simulink model "PV_CHAR"  (R2024a)
settings: Solver=VariableStepAuto  StartTime=0.0  StopTime=5  RelTol=1e-3
libraries: spsDiodeLib x12, spsPVArrayLib x12, spsControlledVoltageSourceLib x2, spsCurrentMeasurementLib x2, simulink x2, spsVoltageMeasurementLib x2, spspowerguiLib x1
settings Model: Creator=sarve  LastModifiedBy=Aswin

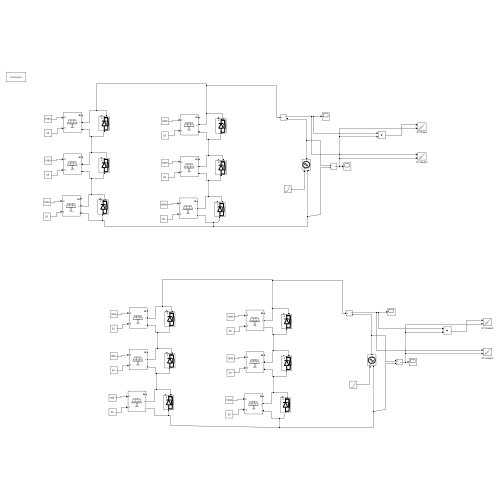
[thumbnail: Simulink's stored preview of the top-level diagram]
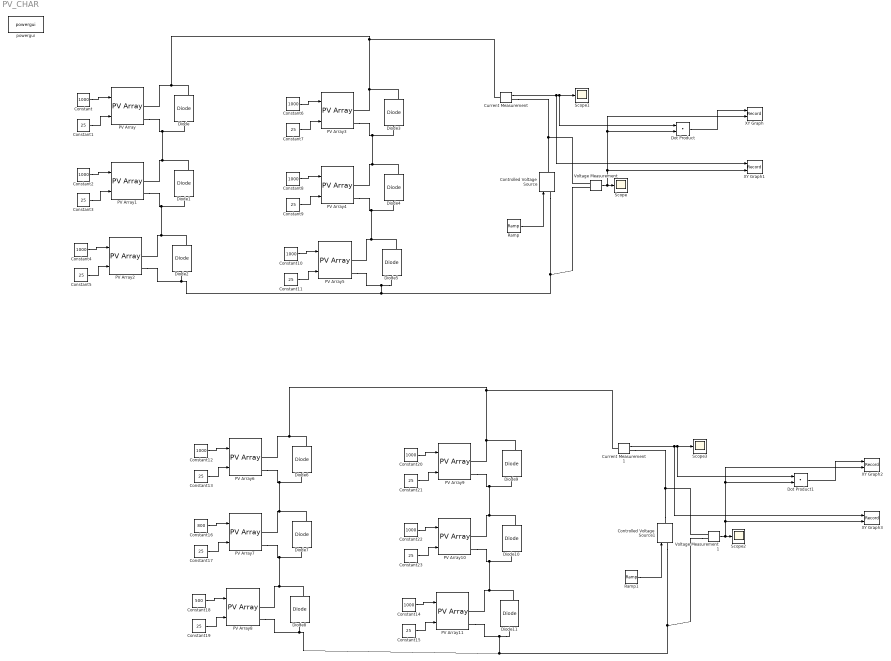
== system PV_CHAR ==
  Constant{,2,4,6,8,10,12,14,20,22} (10 alike) : Constant  Value=1000
  Constant{1,3,5,7,9,11,13,15,17,19,21,23} (12 alike) : Constant  Value=25
  Constant16 : Constant  Value=800
  Constant18 : Constant  Value=500
  Controlled Voltage Source : spsControlledVoltageSourceLib/Controlled Voltage Source  Initialize=on  Source_Type=AC  Amplitude=0  Phase=0  Frequency=0  Measurements=None
  Controlled Voltage Source1 : spsControlledVoltageSourceLib/Controlled Voltage Source  Initialize=on  Source_Type=AC  Amplitude=0  Phase=0  Frequency=0  Measurements=None
  Current Measurement : spsCurrentMeasurementLib/Current Measurement  PhasorSimulation=off  OutputType=Complex  PSBequivalent=0
  Current Measurement1 : spsCurrentMeasurementLib/Current Measurement  PhasorSimulation=off  OutputType=Complex  PSBequivalent=0
  Diode{,1..11} (12 alike) : spsDiodeLib/Diode  Ron=0.001  Lon=0  Vf=0.8  IC=0  UseSnubber=0  Rs=500  Cs=250e-9  Measurements=on
  Dot Product : DotProduct  OutDataTypeStr=Inherit: Inherit via internal rule
  Dot Product1 : DotProduct  OutDataTypeStr=Inherit: Inherit via internal rule
  PV Array{,1..11} (12 alike) : spsPVArrayLib/PV Array  Npar=40  Nser=10  PlotType=array @ 1000 W/m2 & specified temperatures  S_vec="[ 1000  500  100 ]"  Temp_C_vec="[ 45 25  ]"  ModuleName=User-defined  PlotWhenSelected=off  Pm=213.15  Ncell=60  Voc=36.3  Isc=7.84  Vm=29  Im=7.35  beta_Voc_pc=-0.36099  alpha_Isc_pc=0.102  beta_Voc=-0.13104  alpha_Isc=0.0079968  IL=7.8654  I0=2.9273e-10  nI=0.98119  Rsh=313.0553  Rs=0.39381  RobustModel=off  RobustCellTemperature=313.3991  BAL=on  Tc=1e-6  Tfilter=5e-5
  Ramp : simulink/Sources/Ramp  slope=36.3*3*2  start=0  InitialOutput=0
  Ramp1 : simulink/Sources/Ramp  slope=36.3*3*2  start=0  InitialOutput=0
  Scope{,1..3} (4 alike) : Scope
  Voltage Measurement : spsVoltageMeasurementLib/Voltage Measurement  PhasorSimulation=off  OutputType=Complex  PSBequivalent=0
  Voltage Measurement1 : spsVoltageMeasurementLib/Voltage Measurement  PhasorSimulation=off  OutputType=Complex  PSBequivalent=0
  XY Graph : Record  FileSettingsInternal="{\"entries\":[{\"content\":{\"excelSettings\":{\"content\":{},\"type\":\"Streamout.ExcelSettings\"}},\"type\":\"Streamout.FileSettingStorage\",\"uuid\":\"\"}],\"packageUris\":[\"http:\\/\\/schema.mathworks.com\\/mf0\\/streamout_blocks\\/R2020a\"],\"version\":\"1.0\"}"  Layout=[1 1]  SignalsInternal="{\"entries\":[{\"content\":{\"signals\":[{\"content\":{\"blockPath\":[],\"dimensions\":[1],\"domain\":\"\",\"lineColor\":\"#64d413\",\"lineWidth\":2,\"plots\":[ 1 ],\"port\":1,\"signalID\":1,\"signalName\":\"Dot Product\"},\"type\":\"RecordBlkView.Signal\",\"uuid\":\"\"},{\"content\":{\"blockPath\":[],\"dimensions\":[1],\"domain\":\"\",\"lineColor\":\"#ff13a6\",\"lineWidth\":2,\"plots\":[ 1 ],\"port\":2,\"signalID\":2,\"signalName\":\"Voltage Measurement\"},\"type\":\"RecordBlkView.Signal\",\"uuid\":\"\"}]},\"type\":\"RecordBlkView.InputSignals\",\"uuid\":\"\"}],\"packageUris\":[\"http:\\/\\/schema.mathworks.com\\/mf0\\/streamout_blocks\\/R2020a\"],\"version\":\"1.0\"}"  VisualizationBindings="{\"xyplotplugin\":{\"info\":[{\"series\":[{\"bindingParametersList\":[{\"parameter\":\"X-Axis\",\"signalID\":2,\"signalName\":\"Voltage Measurement\"},{\"parameter\":\"Y-Axis\",\"signalID\":1,\"signalName\":\"Dot Product\"}],\"seriesID\":0}],\"subplotID\":1}]}}"  CompatibilityTag=XY
  XY Graph1 : Record  FileSettingsInternal="{\"entries\":[{\"content\":{\"excelSettings\":{\"content\":{},\"type\":\"Streamout.ExcelSettings\"}},\"type\":\"Streamout.FileSettingStorage\",\"uuid\":\"\"}],\"packageUris\":[\"http:\\/\\/schema.mathworks.com\\/mf0\\/streamout_blocks\\/R2020a\"],\"version\":\"1.0\"}"  Layout=[1 1]  SignalsInternal="{\"entries\":[{\"content\":{\"signals\":[{\"content\":{\"blockPath\":[],\"dimensions\":[1],\"domain\":\"\",\"lineColor\":\"#0072bd\",\"lineWidth\":2,\"plots\":[ 1 ],\"port\":1,\"signalID\":1,\"signalName\":\"Current Measurement\"},\"type\":\"RecordBlkView.Signal\",\"uuid\":\"\"},{\"content\":{\"blockPath\":[],\"dimensions\":[1],\"domain\":\"\",\"lineColor\":\"#d95319\",\"lineWidth\":2,\"plots\":[ 1 ],\"port\":2,\"signalID\":2,\"signalName\":\"Voltage Measurement\"},\"type\":\"RecordBlkView.Signal\",\"uuid\":\"\"}]},\"type\":\"RecordBlkView.InputSignals\",\"uuid\":\"\"}],\"packageUris\":[\"http:\\/\\/schema.mathworks.com\\/mf0\\/streamout_blocks\\/R2020a\"],\"version\":\"1.0\"}"  VisualizationBindings="{\"xyplotplugin\":{\"info\":[{\"series\":[{\"bindingParametersList\":[{\"parameter\":\"X-Axis\",\"signalID\":2,\"signalName\":\"Voltage Measurement\"},{\"parameter\":\"Y-Axis\",\"signalID\":1,\"signalName\":\"Current Measurement\"}],\"seriesID\":0}],\"subplotID\":1}]}}"  CompatibilityTag=XY
  XY Graph2 : Record  FileSettingsInternal="{\"entries\":[{\"content\":{\"excelSettings\":{\"content\":{},\"type\":\"Streamout.ExcelSettings\"}},\"type\":\"Streamout.FileSettingStorage\",\"uuid\":\"\"}],\"packageUris\":[\"http:\\/\\/schema.mathworks.com\\/mf0\\/streamout_blocks\\/R2020a\"],\"version\":\"1.0\"}"  Layout=[1 1]  SignalsInternal="{\"entries\":[{\"content\":{\"signals\":[{\"content\":{\"blockPath\":[],\"dimensions\":[1],\"domain\":\"\",\"lineColor\":\"#edb120\",\"lineWidth\":2,\"plots\":[ 1 ],\"port\":1,\"signalID\":1,\"signalName\":\"Dot Product1\"},\"type\":\"RecordBlkView.Signal\",\"uuid\":\"\"},{\"content\":{\"blockPath\":[],\"dimensions\":[1],\"domain\":\"\",\"lineColor\":\"#7e2f8e\",\"lineWidth\":2,\"plots\":[ 1 ],\"port\":2,\"signalID\":2,\"signalName\":\"Voltage Measurement1\"},\"type\":\"RecordBlkView.Signal\",\"uuid\":\"\"}]},\"type\":\"RecordBlkView.InputSignals\",\"uuid\":\"\"}],\"packageUris\":[\"http:\\/\\/schema.mathworks.com\\/mf0\\/streamout_blocks\\/R2020a\"],\"version\":\"1.0\"}"  VisualizationBindings="{\"xyplotplugin\":{\"info\":[{\"series\":[{\"bindingParametersList\":[{\"parameter\":\"X-Axis\",\"signalID\":2,\"signalName\":\"Voltage Measurement1\"},{\"parameter\":\"Y-Axis\",\"signalID\":1,\"signalName\":\"Dot Product1\"}],\"seriesID\":0}],\"subplotID\":1}]}}"  CompatibilityTag=XY
  XY Graph3 : Record  FileSettingsInternal="{\"entries\":[{\"content\":{\"excelSettings\":{\"content\":{},\"type\":\"Streamout.ExcelSettings\"}},\"type\":\"Streamout.FileSettingStorage\",\"uuid\":\"\"}],\"packageUris\":[\"http:\\/\\/schema.mathworks.com\\/mf0\\/streamout_blocks\\/R2020a\"],\"version\":\"1.0\"}"  Layout=[1 1]  SignalsInternal="{\"entries\":[{\"content\":{\"signals\":[{\"content\":{\"blockPath\":[],\"dimensions\":[1],\"domain\":\"\",\"lineColor\":\"#a2142f\",\"plots\":[ 1 ],\"port\":1,\"signalID\":1,\"signalName\":\"Current Measurement1\"},\"type\":\"RecordBlkView.Signal\",\"uuid\":\"\"},{\"content\":{\"blockPath\":[],\"dimensions\":[1],\"domain\":\"\",\"lineColor\":\"#4dbeee\",\"lineWidth\":2,\"port\":2,\"signalID\":2,\"signalName\":\"Voltage Measurement1\"},\"type\":\"RecordBlkView.Signal\",\"uuid\":\"\"}]},\"type\":\"RecordBlkView.InputSignals\",\"uuid\":\"\"}],\"packageUris\":[\"http:\\/\\/schema.mathworks.com\\/mf0\\/streamout_blocks\\/R2020a\"],\"version\":\"1.0\"}"  VisualizationBindings="{\"xyplotplugin\":{\"info\":[{\"series\":[{\"bindingParametersList\":[{\"parameter\":\"Y-Axis\",\"signalID\":1,\"signalName\":\"Current Measurement1\"}],\"seriesID\":0}],\"subplotID\":1}]}}"  CompatibilityTag=XY
  powergui : spspowerguiLib/powergui  Priority=1  SimulationMode=Continuous  SampleTime=50e-6  frequency=60  Iterations=50  frequencyindice=0  Pbase=100e6  ErrMax=1e-4  UnitsV=kV  UnitsW=MW  buscounter=0  FunctionMessages=off  echomessages=off  EnableUseOfTLC=off  CurrentSourceSwitches=off  DisableSnubberDevices=off  DisableRonSwitches=off  DisableVfSwitches=off  DisplayEquations=off  AutomaticDiscreteSolvers=off  SolverType=Tustin/Backward Euler (TBE)  Interpol=off  ExternalGateDelay=off  methode=off  Ts=100  x0status=blocks  SPID=on  SwTol=0  HookPort=off  NonlinearTolerance=1e-4  nMaxIteration=100  ContinueOnMaxIteration=off  RestoreLinks=warning  ResistiveCurrentMeasurement=off  Frange=[0:2:500]  Ylog=off  Xlog=on  ShowGrid=off  save=off  variable=ZData  structure=0  ZoomFFT=off  StartTime=0.0  cycles=1  DisplayStyle=1  fundamental=60  FreqAxis=off  MaxFrequency=1000  frequencyindicesteady=1  RmsSteady=1  display=off
  wires:
  Constant/1 -> PV Array/1
  Constant1/1 -> PV Array/2
  Constant2/1 -> PV Array1/1
  Constant3/1 -> PV Array1/2
  Constant4/1 -> PV Array2/1
  Constant5/1 -> PV Array2/2
  Ramp/1 -> Controlled Voltage Source/1
  Voltage Measurement/1 -> XY Graph/2, Dot Product/2, XY Graph1/2, Scope/1
  Current Measurement/1 -> XY Graph1/1, Dot Product/1, Scope1/1
  Constant9/1 -> PV Array4/2
  Constant8/1 -> PV Array4/1
  Constant6/1 -> PV Array3/1
  Constant10/1 -> PV Array5/1
  Constant11/1 -> PV Array5/2
  Constant7/1 -> PV Array3/2
  Dot Product/1 -> XY Graph/1
  Constant23/1 -> PV Array10/2
  Constant22/1 -> PV Array10/1
  Dot Product1/1 -> XY Graph2/1
  Constant15/1 -> PV Array11/2
  Constant21/1 -> PV Array9/2
  Current Measurement1/1 -> XY Graph3/1, Dot Product1/1, Scope3/1
  Constant20/1 -> PV Array9/1
  Constant17/1 -> PV Array7/2
  Constant16/1 -> PV Array7/1
  Constant18/1 -> PV Array8/1
  Constant12/1 -> PV Array6/1
  Constant13/1 -> PV Array6/2
  Constant19/1 -> PV Array8/2
  Constant14/1 -> PV Array11/1
  Ramp1/1 -> Controlled Voltage Source1/1
  Voltage Measurement1/1 -> XY Graph2/2, Dot Product1/2, XY Graph3/2, Scope2/1
  connections:
  PV Array/RConn2 -- PV Array1/RConn1 -- Diode1/RConn1 -- Diode/LConn1
  PV Array1/RConn2 -- PV Array2/RConn1 -- Diode2/RConn1 -- Diode1/LConn1
  Current Measurement/RConn1 -- Voltage Measurement/LConn1 -- Controlled Voltage Source/RConn1
  Diode4/RConn1 -- Diode3/LConn1 -- PV Array3/RConn2 -- PV Array4/RConn1
  PV Array4/RConn2 -- PV Array5/RConn1 -- Diode5/RConn1 -- Diode4/LConn1
  Controlled Voltage Source/LConn1 -- PV Array2/RConn2 -- Diode2/LConn1 -- Diode5/LConn1 -- PV Array5/RConn2 -- Voltage Measurement/LConn2
  Diode/RConn1 -- PV Array3/RConn1 -- Diode3/RConn1 -- Current Measurement/LConn1 -- PV Array/RConn1
  Diode10/RConn1 -- Diode9/LConn1 -- PV Array9/RConn2 -- PV Array10/RConn1
  PV Array10/RConn2 -- PV Array11/RConn1 -- Diode11/RConn1 -- Diode10/LConn1
  Voltage Measurement1/LConn2 -- Controlled Voltage Source1/LConn1 -- PV Array8/RConn2 -- Diode8/LConn1 -- Diode11/LConn1 -- PV Array11/RConn2
  Diode7/RConn1 -- Diode6/LConn1 -- PV Array6/RConn2 -- PV Array7/RConn1
  PV Array7/RConn2 -- PV Array8/RConn1 -- Diode8/RConn1 -- Diode7/LConn1
  Diode6/RConn1 -- PV Array9/RConn1 -- Diode9/RConn1 -- Current Measurement1/LConn1 -- PV Array6/RConn1
  Controlled Voltage Source1/RConn1 -- Current Measurement1/RConn1 -- Voltage Measurement1/LConn1
